simulink model "testrig_AirOilPiston_lib"  (R2026b)
settings: Solver=VariableStepAuto
values from neighbouring files (symbols this model uses):
  Xstraight = [0 0.1 0.2 0.3 0.4 0.5 0.6 0.7 0.8 0.9 1 1.1 ... (7165 elements, 7165x1)]    [testrig_AirOilPiston_roughroad.mat]
  Zstraight = [1479.83533405 1479.80219874 1479.80504396 1479.80808937 1479.81223193 1479.80459058 1479.82104958 1479.81056753 1479.81248059 1479.81165525 1479.82702704 1479.82651781 ... (7165 elements, 7165x1)]    [testrig_AirOilPiston_roughroad.mat]
undefined symbols (not defined in the file or in its folder): Rough
libraries: simulink x5
settings Model: Creator=smiller  LastModifiedBy=smiller

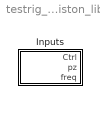
== system testrig_AirOilPiston_lib ==
  Inputs : Subsystem  mask{popup_suspension_stiffness=Soft, popup_rh_test_seq=None, cvd_value=1, popup_roadpz_test_type=Rough, pAmp=1, tPer=4, nCyc=50, nCycSet=1, chirpFreqFinish=10, chirpFreqStart=0.5, chirpTimeFinish=25, chirpTimeStart=5, spdkmh=10, roughTimeStart=5}
      mask prompts: popup_suspension_stiffness "Air Spring Setting"; popup_rh_test_seq "Ride Height Test Sequence"; cvd_value "Damper"; popup_roadpz_test_type "Test Type"; pAmp "Amplitude"; tPer "Period"; nCyc "Number of Cycles per Set"; nCycSet "Number of Cycles to Settle"; chirpFreqFinish "Chirp Freq Finish (Hz)"; chirpFreqStart "Chirp Freq Start (Hz)"; chirpTimeFinish "Chirp Time Finish (sec)"; chirpTimeStart "Chirp Start Delay (sec)"; spdkmh "Speed along Rough Road (km/h)"; roughTimeStart "Settle Time Rough Road (sec)"
      mask init:
      | bh = gcb;
      | softSusp = get_param(bh,'popup_suspension_stiffness');
      | if(strcmp(softSusp,'Soft'))
      |     set_param([bh '/Soft Suspension'],'Value','1');
      | else
      |     set_param([bh '/Soft Suspension'],'Value','0');
      | end
      settings: AttributesFormatString=|
      | Road Height: %<popup_roadpz_test_type>
      | Suspension: %<popup_suspension_stiffness>
      | Ride Height: %<popup_rh_test_seq>
      mask TypeOptions popup_suspension_stiffness: Soft | Stiff
      mask TypeOptions popup_rh_test_seq: Ride Height Test Sequence/popup_test_sequence
      mask TypeOptions cvd_value: PropDamper/Value
      mask TypeOptions popup_roadpz_test_type: Platform Position/popup_signalType
      mask Callback popup_roadpz_test_type:
      | bh = gcb;
      | maskObj = Simulink.Mask.get(bh); % Get the mask object of the current block
      | 
      | % Handles for parameter visibility
      | chFrSt_h  = maskObj.getParameter('chirpFreqStart'); % Get the parameter to hide
      | chFrFi_h  = maskObj.getParameter('chirpFreqFinish'); % Get the parameter to hide
      | chTiSt_h  = maskObj.getParameter('chirpTimeStart'); % Get the parameter to hide
      | chTiFi_h  = maskObj.getParameter('chirpTimeFinish'); % Get the parameter to hide
      | 
      | tPer_h    = maskObj.getParameter('tPer');    % Get the parameter to hide
      | nCycSet_h = maskObj.getParameter('nCycSet'); % Get the parameter to hide
      | nCyc_h    = maskObj.getParameter('nCyc'); % Get the parameter to hide
      | 
      | spdkmh_h   = maskObj.getParameter('spdkmh'); % Get the parameter to hide
      | roughSt_h  = maskObj.getParameter('roughTimeStart'); % Get the parameter to hide
      | 
      | % Check the value of ControlParam
      | controlParamValue = get_param(bh, 'popup_roadpz_test_type');
      | 
      | chFrSt_h.Visible   = 'off';
      | chFrFi_h.Visible   = 'off';
      | chTiFi_h.Visible   = 'off';
      | chTiSt_h.Visible   = 'off';
      | spdkmh_h.Visible   = 'off';
      | roughSt_h.Visible  = 'off';
      | tPer_h.Visible     = 'on';
      | nCycSet_h.Visible  = 'on';
      | nCyc_h.Visible     = 'on';
      | 
      | if(strcmp(controlParamValue, 'Chirp'))
      |     chFrSt_h.Visible  = 'on';
      |     chFrFi_h.Visible  = 'on';
      |     chTiSt_h.Visible  = 'on';
      |     chTiFi_h.Visible  = 'on';
      | 
      |     spdkmh_h.Visible  = 'off';
      |     roughSt_h.Visible  = 'off';
      |     tPer_h.Visible    = 'off';
      |     nCycSet_h.Visible = 'off';
      |     nCyc_h.Visible    = 'off';
      | elseif(strcmp(controlParamValue, 'Rough'))
      |     spdkmh_h.Visible   = 'on';
      |     roughSt_h.Visible  = 'on';
      | 
      |     chFrSt_h.Visible   = 'off';
      |     chFrFi_h.Visible   = 'off';
      |     chTiFi_h.Visible   = 'off';
      |     chTiSt_h.Visible   = 'off';
      |     tPer_h.Visible     = 'off';
      |     nCycSet_h.Visible  = 'off';
      |     nCyc_h.Visible     = 'off';
      | 
      | end
      mask TypeOptions pAmp: Platform Position/pAmp
      mask TypeOptions tPer: Platform Position/tPer
      mask TypeOptions nCyc: Platform Position/nCyc
      mask TypeOptions nCycSet: Platform Position/nCycSet
      mask TypeOptions chirpFreqFinish: Platform Position/chirpFreqFinish
      mask TypeOptions chirpFreqStart: Platform Position/chirpFreqStart
      mask TypeOptions chirpTimeFinish: Platform Position/chirpTimeFinish
      mask TypeOptions chirpTimeStart: Platform Position/chirpTimeStart
      mask TypeOptions spdkmh: Platform Position/spdkmh
      mask TypeOptions roughTimeStart: Platform Position/roughTimeStart
      mask DialogControl Container5 Prompt: Control
      mask DialogControl cont_usmp Prompt: Position Input

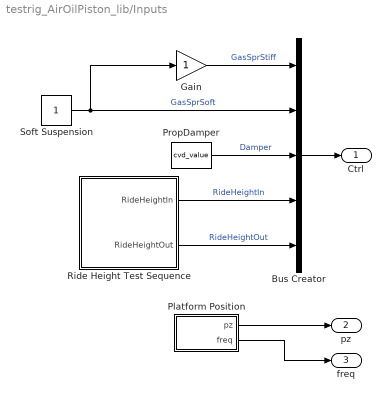
== system testrig_AirOilPiston_lib/Inputs ==
  Bus Creator : BusCreator  Inputs=5
  Gain : Gain
  Platform Position : Subsystem  mask{popup_signalType=Rough, tPer=tPer, chirpFreqStart=chirpFreqStart, chirpFreqFinish=chirpFreqFinish, chirpTimeStart=chirpTimeStart, chirpTimeFinish=chirpTimeFinish, pAmp=pAmp, nCyc=nCyc, nCycSet=nCycSet, spdkmh=spdkmh, roughTimeStart=roughTimeStart}
      mask prompts: popup_signalType "Signal Type"; tPer "Period"; chirpFreqStart "Chirp Freq Start (Hz)"; chirpFreqFinish "Chirp Freq Finish (Hz)"; chirpTimeStart "Chirp Start Delay (sec)"; chirpTimeFinish "Chirp Time Finish (sec)"; pAmp "Amplitude"; nCyc "Number of Cycles per Set"; nCycSet "Number of Cycles to Settle"; spdkmh "Speed along Rough Road (km/h)"; roughTimeStart "Settle Time Rough Road (sec)"
      mask init:
      | bh = gcb;
      | 
      | sigType = get_param(bh,'popup_signalType');
      | set_param([bh '/Velocity Signal'],'LabelModeActiveChoice',sigType)
      | 
      | pVec_time  = [0 tPer/4 tPer/2 3*tPer/4 tPer];
      | pVec_val_Cyc = [0 1 0 -1 0];
      | 
      | sVec_time  = [0 0.05 0.5 0.55 0.95 1]*tPer;
      | sVec_val_Cyc = [0 1 1 0 0 0];
      | 
      | iVec_time    = [0 0.25 0.27 0.29 0.31 0.75  0.77  0.79 0.81 1]*tPer;
      | iVec_val_Cyc = [0 0    1    1    0    0    -1    -1    0    0];
      | 
      | %qVec_time     = [0 tPer/4 tPer/2 3*tPer/4 tPer]*tPer;
      | %qVec_val_Cyc  = [0 1 0 -1 0];
      | 
      | 
      | %aVec_time  = [0 [0 tPer/2 nCyc*tPer+[-1 0]*tPer/2]+nCycSet*tPer];
      | aVec_time  = [0 [0 1e-3 nCyc*tPer+[-1 0]*1e-3]+nCycSet*tPer];
      | 
      | if(strcmp(sigType,'Chirp') || strcmp(sigType,'Rough'))
      |     aVec_value = [1 1 1 1 1];
      | else
      |     aVec_value = [0 0 1 1 0];
      | end
      settings: AttributesFormatString=%<popup_signalType>
      mask TypeOptions popup_signalType: Sine | Triangle | Step | None | Chirp | Rough
      mask Callback popup_signalType:
      | bh = gcb;
      | maskObj = Simulink.Mask.get(bh); % Get the mask object of the current block
      | 
      | % Handles for parameter visibility
      | chFrSt_h  = maskObj.getParameter('chirpFreqStart'); % Get the parameter to hide
      | chFrFi_h  = maskObj.getParameter('chirpFreqFinish'); % Get the parameter to hide
      | chTiSt_h  = maskObj.getParameter('chirpTimeStart'); % Get the parameter to hide
      | chTiFi_h  = maskObj.getParameter('chirpTimeFinish'); % Get the parameter to hide
      | 
      | tPer_h    = maskObj.getParameter('tPer');    % Get the parameter to hide
      | nCycSet_h = maskObj.getParameter('nCycSet'); % Get the parameter to hide
      | nCyc_h    = maskObj.getParameter('nCyc'); % Get the parameter to hide
      | 
      | spdkmh_h  = maskObj.getParameter('spdkmh'); % Get the parameter to hide
      | roughSt_h  = maskObj.getParameter('roughTimeStart'); % Get the parameter to hide
      | 
      | % Check the value of ControlParam
      | controlParamValue = get_param(bh, 'popup_signalType');
      | 
      | chFrSt_h.Visible   = 'off';
      | chFrFi_h.Visible   = 'off';
      | chTiFi_h.Visible   = 'off';
      | chTiSt_h.Visible   = 'off';
      | spdkmh_h.Visible   = 'off';
      | roughSt_h.Visible  = 'off';
      | tPer_h.Visible     = 'on';
      | nCycSet_h.Visible  = 'on';
      | nCyc_h.Visible     = 'on';
      | 
      | if(strcmp(controlParamValue, 'Chirp'))
      |     chFrSt_h.Visible  = 'on';
      |     chFrFi_h.Visible  = 'on';
      |     chTiSt_h.Visible  = 'on';
      |     chTiFi_h.Visible  = 'on';
      | 
      |     spdkmh_h.Visible  = 'off';
      |     roughSt_h.Visible  = 'off';
      |     tPer_h.Visible    = 'off';
      |     nCycSet_h.Visible = 'off';
      |     nCyc_h.Visible    = 'off';
      | elseif(strcmp(controlParamValue, 'Rough'))
      |     spdkmh_h.Visible   = 'on';
      |     roughSt_h.Visible  = 'on';
      | 
      |     chFrSt_h.Visible   = 'off';
      |     chFrFi_h.Visible   = 'off';
      |     chTiFi_h.Visible   = 'off';
      |     chTiSt_h.Visible   = 'off';
      | 
      |     tPer_h.Visible     = 'off';
      |     nCycSet_h.Visible  = 'off';
      |     nCyc_h.Visible     = 'off';
      | 
      | end
  PropDamper : Constant  Value=cvd_value
  Ride Height Test Sequence : Subsystem  Variant=on  VariantControlMode=label  VariantControl=Pulse Sequence A  LabelModeActiveChoice=None  mask{popup_test_sequence=None}
      mask prompts: popup_test_sequence "Test Sequence"
      mask init:
      | bh = gcb;
      | seqOpt = get_param(bh,'popup_test_sequence');
      | set_param(gcb,'LabelModeActiveChoice',seqOpt);
      mask TypeOptions popup_test_sequence: None | Pulse Sequence A
  Soft Suspension : Constant
  Ctrl : Outport
  pz : Outport  Port=2
  freq : Outport  Port=3
  wires:
  PropDamper/1 -> Bus Creator/3  "Damper"
  Gain/1 -> Bus Creator/1  "GasSprStiff"
  Soft Suspension/1 -> Gain/1, Bus Creator/2  "GasSprSoft"
  Bus Creator/1 -> Ctrl/1
  Platform Position/1(pz) -> pz/1
  Ride Height Test Sequence/1(RideHeightIn) -> Bus Creator/4  "RideHeightIn"
  Ride Height Test Sequence/2(RideHeightOut) -> Bus Creator/5  "RideHeightOut"
  Platform Position/2(freq) -> freq/1

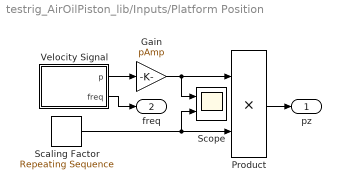
== system testrig_AirOilPiston_lib/Inputs/Platform Position ==
  Gain : Gain  Gain=pAmp
  Product : Product
  Scaling Factor : simulink/Sources/Repeating Sequence  rep_seq_t=aVec_time  rep_seq_y=aVec_value
  Scope : Scope  NumInputPorts=2
      settings: ActiveDisplayYMinimum=-0.015  ActiveDisplayYMaximum=0.135
  Velocity Signal : Subsystem  Variant=on  VariantControlMode=label  VariantControl=Sine  LabelModeActiveChoice=Rough
  pz : Outport
  freq : Outport  Port=2
  wires:
  Scaling Factor/1 -> Scope/2, Product/2
  Product/1 -> pz/1
  Velocity Signal/1(p) -> Gain/1
  Gain/1 -> Product/1, Scope/1
  Velocity Signal/2(freq) -> freq/1

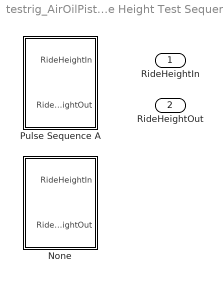
== system testrig_AirOilPiston_lib/Inputs/Ride Height Test Sequence ==
  None : Subsystem  VariantControl=None
  Pulse Sequence A : Subsystem  VariantControl=Pulse Sequence A
  RideHeightIn : Outport
  RideHeightOut : Outport  Port=2

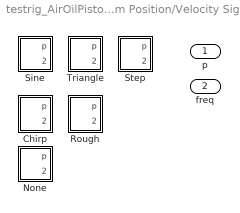
== system testrig_AirOilPiston_lib/Inputs/Platform Position/Velocity Signal ==
  Chirp : Subsystem  VariantControl=Chirp
  None : Subsystem  VariantControl=None
  Rough : Subsystem  VariantControl=Rough
  Sine : Subsystem  VariantControl=Sine
  Step : Subsystem  VariantControl=Step
  Triangle : Subsystem  VariantControl=Triangle
  p : Outport
  freq : Outport  Port=2

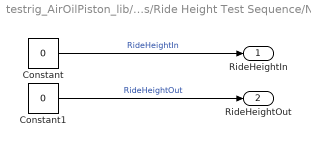
== system testrig_AirOilPiston_lib/Inputs/Ride Height Test Sequence/None ==
  Constant : Constant  Value=0
  Constant1 : Constant  Value=0
  RideHeightIn : Outport
  RideHeightOut : Outport  Port=2
  wires:
  Constant/1 -> RideHeightIn/1  "RideHeightIn"
  Constant1/1 -> RideHeightOut/1  "RideHeightOut"

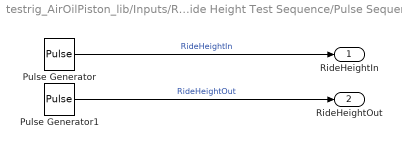
== system testrig_AirOilPiston_lib/Inputs/Ride Height Test Sequence/Pulse Sequence A ==
  Pulse Generator : DiscretePulseGenerator  PulseType=Time based  Amplitude=0.15  Period=10  PulseWidth=5  PhaseDelay=2
  Pulse Generator1 : DiscretePulseGenerator  PulseType=Time based  Amplitude=0.3  Period=10  PulseWidth=5  PhaseDelay=7
  RideHeightIn : Outport
  RideHeightOut : Outport  Port=2
  wires:
  Pulse Generator1/1 -> RideHeightOut/1  "RideHeightOut"
  Pulse Generator/1 -> RideHeightIn/1  "RideHeightIn"

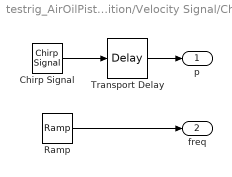
== system testrig_AirOilPiston_lib/Inputs/Platform Position/Velocity Signal/Chirp ==
  Chirp Signal : simulink/Sources/Chirp Signal  f1=chirpFreqStart  T=chirpTimeFinish  f2=chirpFreqFinish
  Ramp : simulink/Sources/Ramp  slope=(chirpFreqFinish-chirpFreqStart)/(chirpTimeFinish)  start=chirpTimeStart  InitialOutput=chirpFreqStart
  Transport Delay : TransportDelay  DelayTime=chirpTimeStart  BufferSize=34816
  p : Outport
  freq : Outport  Port=2
  wires:
  Chirp Signal/1 -> Transport Delay/1
  Transport Delay/1 -> p/1
  Ramp/1 -> freq/1

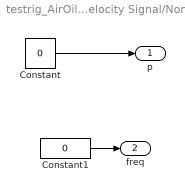
== system testrig_AirOilPiston_lib/Inputs/Platform Position/Velocity Signal/None ==
  Constant : Constant  Value=0
  Constant1 : Constant  Value=0
  p : Outport
  freq : Outport  Port=2
  wires:
  Constant/1 -> p/1
  Constant1/1 -> freq/1

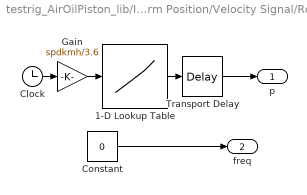
== system testrig_AirOilPiston_lib/Inputs/Platform Position/Velocity Signal/Rough ==
  1-D Lookup Table : Lookup_n-D  NumberOfTableDimensions=1  BreakpointsForDimension1=Xstraight-Xstraight(1)  Table=Zstraight-Zstraight(1)  InternalRulePriority=Speed  RndMeth=Simplest
  Clock : Clock
  Constant : Constant  Value=0
  Gain : Gain  Gain=spdkmh/3.6
  Transport Delay : TransportDelay  DelayTime=roughTimeStart  BufferSize=34816
  p : Outport
  freq : Outport  Port=2
  wires:
  Constant/1 -> freq/1
  Transport Delay/1 -> p/1
  Clock/1 -> Gain/1
  Gain/1 -> 1-D Lookup Table/1
  1-D Lookup Table/1 -> Transport Delay/1

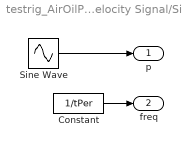
== system testrig_AirOilPiston_lib/Inputs/Platform Position/Velocity Signal/Sine ==
  Constant : Constant  Value=1/tPer
  Sine Wave : Sin  Bias=1  Frequency=2*pi/tPer  Phase=-pi/2  SampleTime=0
  p : Outport
  freq : Outport  Port=2
  wires:
  Sine Wave/1 -> p/1
  Constant/1 -> freq/1

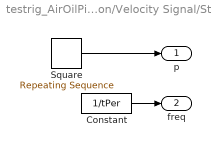
== system testrig_AirOilPiston_lib/Inputs/Platform Position/Velocity Signal/Step ==
  Constant : Constant  Value=1/tPer
  Square : simulink/Sources/Repeating Sequence  rep_seq_t=sVec_time  rep_seq_y=sVec_val_Cyc
  p : Outport
  freq : Outport  Port=2
  wires:
  Square/1 -> p/1
  Constant/1 -> freq/1

== system testrig_AirOilPiston_lib/Inputs/Platform Position/Velocity Signal/Triangle ==
  Constant : Constant  Value=1/tPer
  Triangle : simulink/Sources/Repeating Sequence  rep_seq_t=pVec_time  rep_seq_y=pVec_val_Cyc
  p : Outport
  freq : Outport  Port=2
  wires:
  Triangle/1 -> p/1
  Constant/1 -> freq/1
